simulink model "csd_final_project"  (R2025b)
settings: Solver=VariableStepAuto  StartTime=0.0  StopTime=10.0  RelTol=1e-3
undefined symbols (not defined in the file or in its folder): p, x0
settings Model: Creator=jacobotellop  LastModifiedBy=jacobotellop

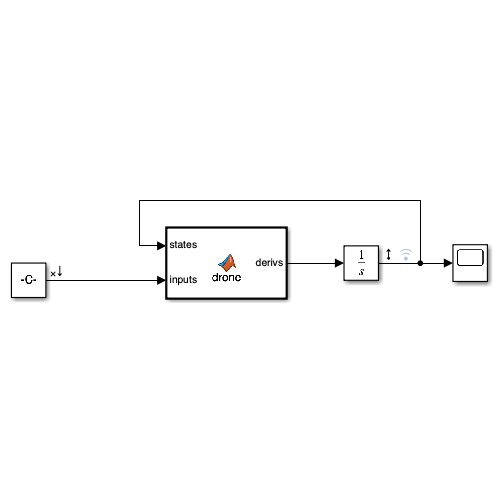
[thumbnail: Simulink's stored preview of the top-level diagram]
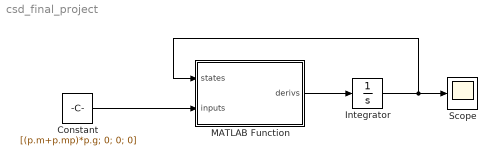
== system csd_final_project ==
  Constant : Constant  Value=[(p.m+p.mp)*p.g; 0; 0; 0]
  Integrator : Integrator  InitialCondition=x0
  MATLAB Function : MATLAB Function  TreatAsAtomicUnit=on
  Scope : Scope
      settings: ActiveDisplayYMinimum=-9.5030918336607108E-11  ActiveDisplayYMaximum=1.9478536826330453E-10
  wires:
  Constant/1 -> MATLAB Function/2(inputs)
  MATLAB Function/1(derivs) -> Integrator/1
  Integrator/1 -> MATLAB Function/1(states), Scope/1

== matlab function csd_final_project/MATLAB Function ==
  data: states input; derivs output; inputs input; p parameter
function derivs = drone(states, inputs, p)

xd    = states(4:6);  
phi   = states(7); 
theta = states(8); 
psi   = states(9);
nu    = states(10:12); 
al    = states(13); 
ald   = states(14);
uT    = inputs(1);  
tau   = inputs(2:4);
M     = p.m + p.mp;

F  = Rot(psi,theta,phi)*[0;0;uT];                       % thrust in inertial frame
c = cos(al); 
s = sin(al);

Minv = [p.m+p.mp*c^2, -p.mp*s*c; -p.mp*s*c, p.m+p.mp*s^2]/(p.m*M);

acc = Minv*([F(1);F(3)] - p.kD*[xd(1);xd(3)] + p.mp*(p.ell*ald^2 - p.g*c)*[s;c] + [0;-p.m*p.g]);
xdd = [acc(1); (F(2)-p.kD*xd(2))/p.m; acc(2)];
add = (-xdd(1)*c + xdd(3)*s + p.g*s)/p.ell;            

I = diag([p.Ixx p.Iyy p.Izz]);
nud    = I\(tau - cross(nu, I*nu));
etadot = Winv(theta,phi)*nu;

derivs = [xd; xdd; etadot; nud; ald; add];
end

function R = Rot(psi,th,ph)
Rz=[cos(psi) -sin(psi) 0; sin(psi) cos(psi) 0; 0 0 1];
Ry=[cos(th) 0 sin(th); 0 1 0; -sin(th) 0 cos(th)];
Rx=[1 0 0; 0 cos(ph) -sin(ph); 0 sin(ph) cos(ph)];
R=Rz*Ry*Rx;
end

function Wi = Winv(th,ph)
Wi=[1 sin(ph)*tan(th) cos(ph)*tan(th); 0 cos(ph) -sin(ph); 0 sin(ph)/cos(th) cos(ph)/cos(th)];
end
